simulink model "Template_v5_0_0_2026a_Linear"  (R2026a)
settings: Solver=ode4  StopTime=tsim  FixedStep=baseRate  RelTol=1e-6  AbsTol=1e-6
PreLoadFcn:
  | spot.buses.define;
  | if ~exist('simMode', 'var'), simMode = 1; end
InitFcn:
  | spot.buses.define;
  | if ~exist('simMode', 'var'), simMode = 1; end
values from neighbouring files (symbols this model uses):
  customControllerParamsBLACK = struct('unused', 0)    [SPOT_User_Parameters.m]
  customControllerParamsBLUE = struct('unused', 0)    [SPOT_User_Parameters.m]
  customControllerParamsRED = struct('unused', 0)    [SPOT_User_Parameters.m]
  customPlannerParamsBLACK = struct('unused', 0)    [SPOT_User_Parameters.m]
  customPlannerParamsBLUE = struct('unused', 0)    [SPOT_User_Parameters.m]
  customPlannerParamsRED = struct('unused', 0)    [SPOT_User_Parameters.m]
undefined symbols (not defined in the file or in its folder): baseRate, BLACK, BLUE, dataRate, DiscIntNeverNeededParam, F_thrusters_BLACK, F_thrusters_BLUE, F_thrusters_RED, home_states_BLACK, home_states_BLUE, home_states_RED, IBLACK, IBLUE, init_states_BLACK, init_states_BLUE, init_states_RED, IRED, K_BLACK, K_BLUE, K_RED, mBLACK, mBLUE, mRED, phase, Phase0_End, Phase1_End, Phase2_End, Phase3_End, Phase4_End, Phase5_End, PWMFreq, RED, tableDamping_BLACK, tableDamping_BLUE, tableDamping_RED, tableSlope, thrust_decay_BLACK, thrust_decay_BLUE, thrust_decay_RED, thruster_dist2CG_BLACK, thruster_dist2CG_BLUE, thruster_dist2CG_RED, time, xLength, yLength
libraries: nvidiaCommlib x1
(part 2 of 2)

== matlab function Template_v5_0_0_2026a_Linear/Plant or Hardware/Simulation/Chaser Plant/callPlatformDynamics ==
  data: forces input; position input; velocity input; floating input; acceleration output; mass parameter; inertia parameter; tableSlope parameter; tableDamping parameter
function acceleration  = callPlatformDynamics(forces, position, velocity,...
    floating, mass, inertia, tableSlope, tableDamping)

    [acceleration] = spot.dynamics.platformDynamics(forces, position,...
        velocity, floating, mass, inertia, tableSlope, tableDamping);
    
end

== matlab function Template_v5_0_0_2026a_Linear/Controllers/Chaser Controller/callController ==
  data: controllerChoice input; state input; setpoint input; controls output; context input Bus: SpotBus; K parameter; customParams parameter
function controls = callController(controllerChoice, state, setpoint, context, K, customParams)
    %CALLCONTROLLER Run the selected control law for one spacecraft.
    %   controllerChoice  1 default LQR, 2 custom, anything else thrusters off
    
    switch controllerChoice
        case 1
            controls = spot.control.defaultController(state, setpoint, K);
        case 2
            controls = spot.control.customController(state, setpoint, context, customParams);
        otherwise
            controls = zeros(3, 1);     % thrusters off
    end
end

== matlab function Template_v5_0_0_2026a_Linear/Mixers/Chaser Mixer/callMixer ==
  data: duty output; controls input; state input; thrusterDist parameter; thrust parameter; PWMFreq parameter; decayPerValve parameter
function duty = callMixer(controls, state, thrusterDist, thrust, PWMFreq, decayPerValve)

    duty = spot.control.allocateThrusters(controls, state.pose(3), thrusterDist, thrust, decayPerValve);
    duty = spot.control.dropShortPulses(duty, PWMFreq);

end

== matlab function Template_v5_0_0_2026a_Linear/Plant or Hardware/Simulation/Chaser Plant/Model Thrusters/callThrusterForces ==
  data: duty input; pose input; thrusterDist parameter; thrust parameter; forces output; decayPerValve parameter
function forces = callThrusterForces(duty, pose, thrusterDist, thrust, decayPerValve)

    forces = spot.dynamics.thrusterForces(duty, pose(3), thrusterDist, thrust, decayPerValve);

end

== matlab function Template_v5_0_0_2026a_Linear/Path Planners/Chaser Planner/callPlanner ==
  data: plannerChoice input; state input Bus: PlatformState; setpoint output Bus: Setpoint; goal input; previousGoal input; context input; maxSpeed parameter; maxTurnRate parameter; horizon parameter; customParams parameter; baseRate parameter
function setpoint = callPlanner(plannerChoice, state, goal, previousGoal, context, maxSpeed, maxTurnRate, horizon, customParams, baseRate)
    %CALLPLANNER Run the selected path planner for one spacecraft.
    %   plannerChoice  0 none (the goal is the setpoint), 1 default, 2 custom,
    %                  anything else hold the current pose

    switch plannerChoice
        case 0
            setpoint = spot.guidance.directPlanner(goal, previousGoal, baseRate);
        case 1
            setpoint = spot.guidance.defaultPlanner(state, goal, maxSpeed, maxTurnRate, horizon);
        case 2
            setpoint = spot.guidance.customPlanner(state, goal, context, customParams);
        otherwise
            setpoint.pose = state.pose;         % hold where it is
            setpoint.rate = zeros(3, 1);
    end
end

== matlab function Template_v5_0_0_2026a_Linear/Controllers/Obstacle Controller/callController ==
  data: controllerChoice input; state input; setpoint input; controls output; context input Bus: SpotBus; K parameter; customParams parameter
function controls = callController(controllerChoice, state, setpoint, context, K, customParams)
    %CALLCONTROLLER Run the selected control law for one spacecraft.
    %   controllerChoice  1 default LQR, 2 custom, anything else thrusters off
    
    switch controllerChoice
        case 1
            controls = spot.control.defaultController(state, setpoint, K);
        case 2
            controls = spot.control.customController(state, setpoint, context, customParams);
        otherwise
            controls = zeros(3, 1);     % thrusters off
    end
end

== matlab function Template_v5_0_0_2026a_Linear/Plant or Hardware/Simulation/Target Plant/Model Thrusters/callHoldDuty ==
  data: duty output; newDuty input; previousDuty input; time input; PWMFreq parameter; baseRate parameter
function duty = callHoldDuty(newDuty, previousDuty, time, PWMFreq, baseRate)

    duty = spot.control.holdDuty(newDuty, previousDuty, time, PWMFreq, baseRate);

end

== matlab function Template_v5_0_0_2026a_Linear/Mixers/Target Mixer/callMixer ==
  data: duty output; controls input; state input; thrusterDist parameter; thrust parameter; PWMFreq parameter; decayPerValve parameter
function duty = callMixer(controls, state, thrusterDist, thrust, PWMFreq, decayPerValve)

    duty = spot.control.allocateThrusters(controls, state.pose(3), thrusterDist, thrust, decayPerValve);
    duty = spot.control.dropShortPulses(duty, PWMFreq);

end

== matlab function Template_v5_0_0_2026a_Linear/Plant or Hardware/Simulation/Target Plant/Model Thrusters/callThrusterForces ==
  data: duty input; pose input; thrusterDist parameter; thrust parameter; forces output; decayPerValve parameter
function forces = callThrusterForces(duty, pose, thrusterDist, thrust, decayPerValve)

    forces = spot.dynamics.thrusterForces(duty, pose(3), thrusterDist, thrust, decayPerValve);

end

== matlab function Template_v5_0_0_2026a_Linear/Mixers/Obstacle Mixer/callMixer ==
  data: duty output; controls input; state input; thrusterDist parameter; thrust parameter; PWMFreq parameter; decayPerValve parameter
function duty = callMixer(controls, state, thrusterDist, thrust, PWMFreq, decayPerValve)

    duty = spot.control.allocateThrusters(controls, state.pose(3), thrusterDist, thrust, decayPerValve);
    duty = spot.control.dropShortPulses(duty, PWMFreq);

end

== matlab function Template_v5_0_0_2026a_Linear/Plant or Hardware/Simulation/Target Plant/callMeasureState ==
  data: truePose input; time input; measured output Bus: PlatformState; previousMeasured input Bus: PlatformState; dataRate parameter; baseRate parameter
function measured = callMeasureState(truePose, time, previousMeasured, dataRate, baseRate)

    measured = spot.dynamics.measureState(truePose, previousMeasured, time, dataRate, baseRate);

end
